simulink model "s_c107m32k_vlbi"  (R2018a)
settings: Solver=VariableStepDiscrete  StartTime=0.0  StopTime=(2^15)*10  RelTol=1e-3
undefined symbols (not defined in the file): fft_stages, n_bits_xengs
libraries: xbsIndex_r4 x23049, casper_library_misc x45, xps_library x4, casper_library_scopes x3, simulink x2
(part 151 of 201)

== system s_c107m32k_vlbi/cd_hmc/hmc_delay/ctrl_pol0/add_parity ==
  din : Inport
  Concat : xbsIndex_r4/Concat  num_inputs=2  dbl_ovrd=off  block_type=concat
  Delay1 : xbsIndex_r4/Delay  rst=off  infoeditControl=Selection of Reset will increase slice count due to use of real FFs and instead of SRLs  en=off  latency=3  reg_retiming=on  dbl_ovrd=off  block_type=delay
  Delay2 : xbsIndex_r4/Delay  rst=off  infoeditControl=Selection of Reset will increase slice count due to use of real FFs and instead of SRLs  en=off  latency=1  reg_retiming=on  dbl_ovrd=off  block_type=delay
  bus_expand : Subsystem  AncestorBlock=casper_library_flow_control/bus_expand  mask(bus_expand){mode=divisions of equal size, outputNum=80, outputWidth=1, outputBinaryPt=0, outputArithmeticType=0, show_format=off, outputToWorkspace=off, variablePrefix=out, outputToModelAsWell=on}
      mask prompts: outputNum "Number of outputs:"; outputWidth "Output width:"; outputBinaryPt "Output binary point position:"; outputArithmeticType "Output arithmetic type (ufix=0, fix=1, bool=2):"; show_format "Print format string?"; outputToWorkspace "Output to workspace?"; variablePrefix "Variable name prefix:"; outputToModelAsWell "Output to model as well?"
      mask help:
      | Expands a 'bus' made using a bus_create or Xilinx
      | concat block.
      | The input will be divided into the specified number
      | of outputs with the specified arithmetic types.
      | Divisions are made from most significant bit.
      mask init: same as s_c107m32k_vlbi/bus_expand1
      settings: AttributesFormatString=80 outputs
      mask TypeOptions mode: divisions of equal size | divisions of arbitrary size
      mask Callback mode: bus_expand_callback();
      mask Callback outputWidth: bus_expand_callback();
      mask Callback outputToWorkspace: bus_expand_callback();
  parity : xbsIndex_r4/Logical  logical_function=XOR  inputs=80  en=off  latency=3  precision=Full  arith_type=Unsigned  n_bits=16  bin_pt=0  align_bp=on  dbl_ovrd=off  block_type=logical
  dout : Outport
  wires:
  Concat/1 -> dout/1
  parity/1 -> Concat/1
  Delay1/1 -> Concat/2
  din/1 -> Delay2/1
  bus_expand/70(out11) -> parity/70
  bus_expand/8(out73) -> parity/8
  bus_expand/31(out50) -> parity/31
  bus_expand/24(out57) -> parity/24
  bus_expand/30(out51) -> parity/30
  bus_expand/38(out43) -> parity/38
  bus_expand/61(out20) -> parity/61
  bus_expand/50(out31) -> parity/50
  bus_expand/77(out4) -> parity/77
  bus_expand/4(out77) -> parity/4
  bus_expand/68(out13) -> parity/68
  bus_expand/59(out22) -> parity/59
  bus_expand/65(out16) -> parity/65
  bus_expand/14(out67) -> parity/14
  bus_expand/7(out74) -> parity/7
  bus_expand/44(out37) -> parity/44
  bus_expand/43(out38) -> parity/43
  bus_expand/23(out58) -> parity/23
  bus_expand/22(out59) -> parity/22
  bus_expand/67(out14) -> parity/67
  bus_expand/2(out79) -> parity/2
  bus_expand/48(out33) -> parity/48
  bus_expand/42(out39) -> parity/42
  bus_expand/78(out3) -> parity/78
  bus_expand/58(out23) -> parity/58
  bus_expand/80(lsb_out1) -> parity/80
  bus_expand/72(out9) -> parity/72
  bus_expand/18(out63) -> parity/18
  bus_expand/15(out66) -> parity/15
  bus_expand/17(out64) -> parity/17
  bus_expand/1(msb_out80) -> parity/1
  bus_expand/6(out75) -> parity/6
  bus_expand/47(out34) -> parity/47
  bus_expand/37(out44) -> parity/37
  bus_expand/71(out10) -> parity/71
  bus_expand/73(out8) -> parity/73
  bus_expand/51(out30) -> parity/51
  bus_expand/21(out60) -> parity/21
  bus_expand/13(out68) -> parity/13
  bus_expand/20(out61) -> parity/20
  bus_expand/76(out5) -> parity/76
  bus_expand/57(out24) -> parity/57
  bus_expand/63(out18) -> parity/63
  bus_expand/33(out48) -> parity/33
  bus_expand/75(out6) -> parity/75
  bus_expand/60(out21) -> parity/60
  bus_expand/54(out27) -> parity/54
  bus_expand/28(out53) -> parity/28
  bus_expand/69(out12) -> parity/69
  bus_expand/10(out71) -> parity/10
  bus_expand/32(out49) -> parity/32
  bus_expand/62(out19) -> parity/62
  bus_expand/36(out45) -> parity/36
  bus_expand/64(out17) -> parity/64
  bus_expand/46(out35) -> parity/46
  bus_expand/3(out78) -> parity/3
  bus_expand/56(out25) -> parity/56
  bus_expand/5(out76) -> parity/5
  bus_expand/19(out62) -> parity/19
  bus_expand/74(out7) -> parity/74
  bus_expand/25(out56) -> parity/25
  bus_expand/49(out32) -> parity/49
  bus_expand/11(out70) -> parity/11
  bus_expand/52(out29) -> parity/52
  bus_expand/41(out40) -> parity/41
  bus_expand/79(out2) -> parity/79
  bus_expand/27(out54) -> parity/27
  bus_expand/29(out52) -> parity/29
  bus_expand/26(out55) -> parity/26
  bus_expand/45(out36) -> parity/45
  bus_expand/34(out47) -> parity/34
  bus_expand/12(out69) -> parity/12
  bus_expand/16(out65) -> parity/16
  bus_expand/9(out72) -> parity/9
  bus_expand/55(out26) -> parity/55
  bus_expand/40(out41) -> parity/40
  bus_expand/35(out46) -> parity/35
  bus_expand/39(out42) -> parity/39
  bus_expand/66(out15) -> parity/66
  bus_expand/53(out28) -> parity/53
  Delay2/1 -> Delay1/1, bus_expand/1(bus_in)

== system s_c107m32k_vlbi/cd_hmc/hmc_delay/ctrl_pol1/add_parity ==
  din : Inport
  Concat : xbsIndex_r4/Concat  num_inputs=2  dbl_ovrd=off  block_type=concat
  Delay1 : xbsIndex_r4/Delay  rst=off  infoeditControl=Selection of Reset will increase slice count due to use of real FFs and instead of SRLs  en=off  latency=3  reg_retiming=on  dbl_ovrd=off  block_type=delay
  Delay2 : xbsIndex_r4/Delay  rst=off  infoeditControl=Selection of Reset will increase slice count due to use of real FFs and instead of SRLs  en=off  latency=1  reg_retiming=on  dbl_ovrd=off  block_type=delay
  bus_expand : Subsystem  AncestorBlock=casper_library_flow_control/bus_expand  mask(bus_expand){mode=divisions of equal size, outputNum=80, outputWidth=1, outputBinaryPt=0, outputArithmeticType=0, show_format=off, outputToWorkspace=off, variablePrefix=out, outputToModelAsWell=on}
      mask prompts: outputNum "Number of outputs:"; outputWidth "Output width:"; outputBinaryPt "Output binary point position:"; outputArithmeticType "Output arithmetic type (ufix=0, fix=1, bool=2):"; show_format "Print format string?"; outputToWorkspace "Output to workspace?"; variablePrefix "Variable name prefix:"; outputToModelAsWell "Output to model as well?"
      mask help:
      | Expands a 'bus' made using a bus_create or Xilinx
      | concat block.
      | The input will be divided into the specified number
      | of outputs with the specified arithmetic types.
      | Divisions are made from most significant bit.
      mask init: same as s_c107m32k_vlbi/bus_expand1
      settings: AttributesFormatString=80 outputs
      mask TypeOptions mode: divisions of equal size | divisions of arbitrary size
      mask Callback mode: bus_expand_callback();
      mask Callback outputWidth: bus_expand_callback();
      mask Callback outputToWorkspace: bus_expand_callback();
  parity : xbsIndex_r4/Logical  logical_function=XOR  inputs=80  en=off  latency=3  precision=Full  arith_type=Unsigned  n_bits=16  bin_pt=0  align_bp=on  dbl_ovrd=off  block_type=logical
  dout : Outport
  wires:
  Concat/1 -> dout/1
  parity/1 -> Concat/1
  Delay1/1 -> Concat/2
  din/1 -> Delay2/1
  bus_expand/70(out11) -> parity/70
  bus_expand/8(out73) -> parity/8
  bus_expand/31(out50) -> parity/31
  bus_expand/24(out57) -> parity/24
  bus_expand/30(out51) -> parity/30
  bus_expand/38(out43) -> parity/38
  bus_expand/61(out20) -> parity/61
  bus_expand/50(out31) -> parity/50
  bus_expand/77(out4) -> parity/77
  bus_expand/4(out77) -> parity/4
  bus_expand/68(out13) -> parity/68
  bus_expand/59(out22) -> parity/59
  bus_expand/65(out16) -> parity/65
  bus_expand/14(out67) -> parity/14
  bus_expand/7(out74) -> parity/7
  bus_expand/44(out37) -> parity/44
  bus_expand/43(out38) -> parity/43
  bus_expand/23(out58) -> parity/23
  bus_expand/22(out59) -> parity/22
  bus_expand/67(out14) -> parity/67
  bus_expand/2(out79) -> parity/2
  bus_expand/48(out33) -> parity/48
  bus_expand/42(out39) -> parity/42
  bus_expand/78(out3) -> parity/78
  bus_expand/58(out23) -> parity/58
  bus_expand/80(lsb_out1) -> parity/80
  bus_expand/72(out9) -> parity/72
  bus_expand/18(out63) -> parity/18
  bus_expand/15(out66) -> parity/15
  bus_expand/17(out64) -> parity/17
  bus_expand/1(msb_out80) -> parity/1
  bus_expand/6(out75) -> parity/6
  bus_expand/47(out34) -> parity/47
  bus_expand/37(out44) -> parity/37
  bus_expand/71(out10) -> parity/71
  bus_expand/73(out8) -> parity/73
  bus_expand/51(out30) -> parity/51
  bus_expand/21(out60) -> parity/21
  bus_expand/13(out68) -> parity/13
  bus_expand/20(out61) -> parity/20
  bus_expand/76(out5) -> parity/76
  bus_expand/57(out24) -> parity/57
  bus_expand/63(out18) -> parity/63
  bus_expand/33(out48) -> parity/33
  bus_expand/75(out6) -> parity/75
  bus_expand/60(out21) -> parity/60
  bus_expand/54(out27) -> parity/54
  bus_expand/28(out53) -> parity/28
  bus_expand/69(out12) -> parity/69
  bus_expand/10(out71) -> parity/10
  bus_expand/32(out49) -> parity/32
  bus_expand/62(out19) -> parity/62
  bus_expand/36(out45) -> parity/36
  bus_expand/64(out17) -> parity/64
  bus_expand/46(out35) -> parity/46
  bus_expand/3(out78) -> parity/3
  bus_expand/56(out25) -> parity/56
  bus_expand/5(out76) -> parity/5
  bus_expand/19(out62) -> parity/19
  bus_expand/74(out7) -> parity/74
  bus_expand/25(out56) -> parity/25
  bus_expand/49(out32) -> parity/49
  bus_expand/11(out70) -> parity/11
  bus_expand/52(out29) -> parity/52
  bus_expand/41(out40) -> parity/41
  bus_expand/79(out2) -> parity/79
  bus_expand/27(out54) -> parity/27
  bus_expand/29(out52) -> parity/29
  bus_expand/26(out55) -> parity/26
  bus_expand/45(out36) -> parity/45
  bus_expand/34(out47) -> parity/34
  bus_expand/12(out69) -> parity/12
  bus_expand/16(out65) -> parity/16
  bus_expand/9(out72) -> parity/9
  bus_expand/55(out26) -> parity/55
  bus_expand/40(out41) -> parity/40
  bus_expand/35(out46) -> parity/35
  bus_expand/39(out42) -> parity/39
  bus_expand/66(out15) -> parity/66
  bus_expand/53(out28) -> parity/53
  Delay2/1 -> Delay1/1, bus_expand/1(bus_in)

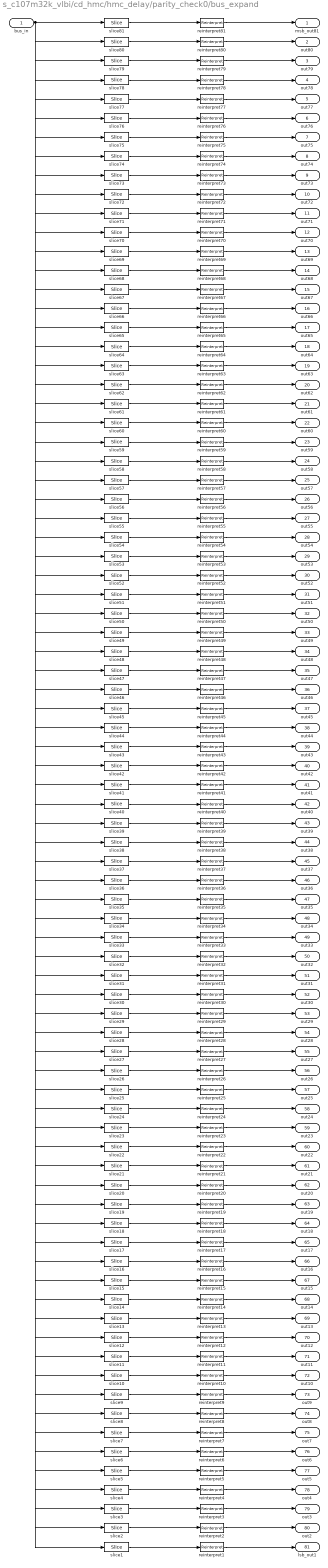
== system s_c107m32k_vlbi/cd_hmc/hmc_delay/parity_check0/bus_expand ==
  bus_in : Inport
  reinterpret{1..81} (81 alike) : xbsIndex_r4/Reinterpret  force_arith_type=on  arith_type=Unsigned  force_bin_pt=on  bin_pt=0  block_type=reinterpret
  slice1 : xbsIndex_r4/Slice  nbits=1  boolean_output=off  mode=Upper Bit Location + Width  bit1=-80  base1=MSB of Input  bit0=0  base0=LSB of Input  dbl_ovrd=off  block_type=slice
  slice10 : xbsIndex_r4/Slice  nbits=1  boolean_output=off  mode=Upper Bit Location + Width  bit1=-71  base1=MSB of Input  bit0=0  base0=LSB of Input  dbl_ovrd=off  block_type=slice
  slice11 : xbsIndex_r4/Slice  nbits=1  boolean_output=off  mode=Upper Bit Location + Width  bit1=-70  base1=MSB of Input  bit0=0  base0=LSB of Input  dbl_ovrd=off  block_type=slice
  slice12 : xbsIndex_r4/Slice  nbits=1  boolean_output=off  mode=Upper Bit Location + Width  bit1=-69  base1=MSB of Input  bit0=0  base0=LSB of Input  dbl_ovrd=off  block_type=slice
  slice13 : xbsIndex_r4/Slice  nbits=1  boolean_output=off  mode=Upper Bit Location + Width  bit1=-68  base1=MSB of Input  bit0=0  base0=LSB of Input  dbl_ovrd=off  block_type=slice
  slice14 : xbsIndex_r4/Slice  nbits=1  boolean_output=off  mode=Upper Bit Location + Width  bit1=-67  base1=MSB of Input  bit0=0  base0=LSB of Input  dbl_ovrd=off  block_type=slice
  slice15 : xbsIndex_r4/Slice  nbits=1  boolean_output=off  mode=Upper Bit Location + Width  bit1=-66  base1=MSB of Input  bit0=0  base0=LSB of Input  dbl_ovrd=off  block_type=slice
  slice16 : xbsIndex_r4/Slice  nbits=1  boolean_output=off  mode=Upper Bit Location + Width  bit1=-65  base1=MSB of Input  bit0=0  base0=LSB of Input  dbl_ovrd=off  block_type=slice
  slice17 : xbsIndex_r4/Slice  nbits=1  boolean_output=off  mode=Upper Bit Location + Width  bit1=-64  base1=MSB of Input  bit0=0  base0=LSB of Input  dbl_ovrd=off  block_type=slice
  slice18 : xbsIndex_r4/Slice  nbits=1  boolean_output=off  mode=Upper Bit Location + Width  bit1=-63  base1=MSB of Input  bit0=0  base0=LSB of Input  dbl_ovrd=off  block_type=slice
  slice19 : xbsIndex_r4/Slice  nbits=1  boolean_output=off  mode=Upper Bit Location + Width  bit1=-62  base1=MSB of Input  bit0=0  base0=LSB of Input  dbl_ovrd=off  block_type=slice
  slice2 : xbsIndex_r4/Slice  nbits=1  boolean_output=off  mode=Upper Bit Location + Width  bit1=-79  base1=MSB of Input  bit0=0  base0=LSB of Input  dbl_ovrd=off  block_type=slice
  slice20 : xbsIndex_r4/Slice  nbits=1  boolean_output=off  mode=Upper Bit Location + Width  bit1=-61  base1=MSB of Input  bit0=0  base0=LSB of Input  dbl_ovrd=off  block_type=slice
  slice21 : xbsIndex_r4/Slice  nbits=1  boolean_output=off  mode=Upper Bit Location + Width  bit1=-60  base1=MSB of Input  bit0=0  base0=LSB of Input  dbl_ovrd=off  block_type=slice
  slice22 : xbsIndex_r4/Slice  nbits=1  boolean_output=off  mode=Upper Bit Location + Width  bit1=-59  base1=MSB of Input  bit0=0  base0=LSB of Input  dbl_ovrd=off  block_type=slice
  slice23 : xbsIndex_r4/Slice  nbits=1  boolean_output=off  mode=Upper Bit Location + Width  bit1=-58  base1=MSB of Input  bit0=0  base0=LSB of Input  dbl_ovrd=off  block_type=slice
  slice24 : xbsIndex_r4/Slice  nbits=1  boolean_output=off  mode=Upper Bit Location + Width  bit1=-57  base1=MSB of Input  bit0=0  base0=LSB of Input  dbl_ovrd=off  block_type=slice
  slice25 : xbsIndex_r4/Slice  nbits=1  boolean_output=off  mode=Upper Bit Location + Width  bit1=-56  base1=MSB of Input  bit0=0  base0=LSB of Input  dbl_ovrd=off  block_type=slice
  slice26 : xbsIndex_r4/Slice  nbits=1  boolean_output=off  mode=Upper Bit Location + Width  bit1=-55  base1=MSB of Input  bit0=0  base0=LSB of Input  dbl_ovrd=off  block_type=slice
  slice27 : xbsIndex_r4/Slice  nbits=1  boolean_output=off  mode=Upper Bit Location + Width  bit1=-54  base1=MSB of Input  bit0=0  base0=LSB of Input  dbl_ovrd=off  block_type=slice
  slice28 : xbsIndex_r4/Slice  nbits=1  boolean_output=off  mode=Upper Bit Location + Width  bit1=-53  base1=MSB of Input  bit0=0  base0=LSB of Input  dbl_ovrd=off  block_type=slice
  slice29 : xbsIndex_r4/Slice  nbits=1  boolean_output=off  mode=Upper Bit Location + Width  bit1=-52  base1=MSB of Input  bit0=0  base0=LSB of Input  dbl_ovrd=off  block_type=slice
  slice3 : xbsIndex_r4/Slice  nbits=1  boolean_output=off  mode=Upper Bit Location + Width  bit1=-78  base1=MSB of Input  bit0=0  base0=LSB of Input  dbl_ovrd=off  block_type=slice
  slice30 : xbsIndex_r4/Slice  nbits=1  boolean_output=off  mode=Upper Bit Location + Width  bit1=-51  base1=MSB of Input  bit0=0  base0=LSB of Input  dbl_ovrd=off  block_type=slice
  slice31 : xbsIndex_r4/Slice  nbits=1  boolean_output=off  mode=Upper Bit Location + Width  bit1=-50  base1=MSB of Input  bit0=0  base0=LSB of Input  dbl_ovrd=off  block_type=slice
  slice32 : xbsIndex_r4/Slice  nbits=1  boolean_output=off  mode=Upper Bit Location + Width  bit1=-49  base1=MSB of Input  bit0=0  base0=LSB of Input  dbl_ovrd=off  block_type=slice
  slice33 : xbsIndex_r4/Slice  nbits=1  boolean_output=off  mode=Upper Bit Location + Width  bit1=-48  base1=MSB of Input  bit0=0  base0=LSB of Input  dbl_ovrd=off  block_type=slice
  slice34 : xbsIndex_r4/Slice  nbits=1  boolean_output=off  mode=Upper Bit Location + Width  bit1=-47  base1=MSB of Input  bit0=0  base0=LSB of Input  dbl_ovrd=off  block_type=slice
  slice35 : xbsIndex_r4/Slice  nbits=1  boolean_output=off  mode=Upper Bit Location + Width  bit1=-46  base1=MSB of Input  bit0=0  base0=LSB of Input  dbl_ovrd=off  block_type=slice
  slice36 : xbsIndex_r4/Slice  nbits=1  boolean_output=off  mode=Upper Bit Location + Width  bit1=-45  base1=MSB of Input  bit0=0  base0=LSB of Input  dbl_ovrd=off  block_type=slice
  slice37 : xbsIndex_r4/Slice  nbits=1  boolean_output=off  mode=Upper Bit Location + Width  bit1=-44  base1=MSB of Input  bit0=0  base0=LSB of Input  dbl_ovrd=off  block_type=slice
  slice38 : xbsIndex_r4/Slice  nbits=1  boolean_output=off  mode=Upper Bit Location + Width  bit1=-43  base1=MSB of Input  bit0=0  base0=LSB of Input  dbl_ovrd=off  block_type=slice
  slice39 : xbsIndex_r4/Slice  nbits=1  boolean_output=off  mode=Upper Bit Location + Width  bit1=-42  base1=MSB of Input  bit0=0  base0=LSB of Input  dbl_ovrd=off  block_type=slice
  slice4 : xbsIndex_r4/Slice  nbits=1  boolean_output=off  mode=Upper Bit Location + Width  bit1=-77  base1=MSB of Input  bit0=0  base0=LSB of Input  dbl_ovrd=off  block_type=slice
  slice40 : xbsIndex_r4/Slice  nbits=1  boolean_output=off  mode=Upper Bit Location + Width  bit1=-41  base1=MSB of Input  bit0=0  base0=LSB of Input  dbl_ovrd=off  block_type=slice
  slice41 : xbsIndex_r4/Slice  nbits=1  boolean_output=off  mode=Upper Bit Location + Width  bit1=-40  base1=MSB of Input  bit0=0  base0=LSB of Input  dbl_ovrd=off  block_type=slice
  slice42 : xbsIndex_r4/Slice  nbits=1  boolean_output=off  mode=Upper Bit Location + Width  bit1=-39  base1=MSB of Input  bit0=0  base0=LSB of Input  dbl_ovrd=off  block_type=slice
  slice43 : xbsIndex_r4/Slice  nbits=1  boolean_output=off  mode=Upper Bit Location + Width  bit1=-38  base1=MSB of Input  bit0=0  base0=LSB of Input  dbl_ovrd=off  block_type=slice
  slice44 : xbsIndex_r4/Slice  nbits=1  boolean_output=off  mode=Upper Bit Location + Width  bit1=-37  base1=MSB of Input  bit0=0  base0=LSB of Input  dbl_ovrd=off  block_type=slice
  slice45 : xbsIndex_r4/Slice  nbits=1  boolean_output=off  mode=Upper Bit Location + Width  bit1=-36  base1=MSB of Input  bit0=0  base0=LSB of Input  dbl_ovrd=off  block_type=slice
  slice46 : xbsIndex_r4/Slice  nbits=1  boolean_output=off  mode=Upper Bit Location + Width  bit1=-35  base1=MSB of Input  bit0=0  base0=LSB of Input  dbl_ovrd=off  block_type=slice
  slice47 : xbsIndex_r4/Slice  nbits=1  boolean_output=off  mode=Upper Bit Location + Width  bit1=-34  base1=MSB of Input  bit0=0  base0=LSB of Input  dbl_ovrd=off  block_type=slice
  slice48 : xbsIndex_r4/Slice  nbits=1  boolean_output=off  mode=Upper Bit Location + Width  bit1=-33  base1=MSB of Input  bit0=0  base0=LSB of Input  dbl_ovrd=off  block_type=slice
  slice49 : xbsIndex_r4/Slice  nbits=1  boolean_output=off  mode=Upper Bit Location + Width  bit1=-32  base1=MSB of Input  bit0=0  base0=LSB of Input  dbl_ovrd=off  block_type=slice
  slice5 : xbsIndex_r4/Slice  nbits=1  boolean_output=off  mode=Upper Bit Location + Width  bit1=-76  base1=MSB of Input  bit0=0  base0=LSB of Input  dbl_ovrd=off  block_type=slice
  slice50 : xbsIndex_r4/Slice  nbits=1  boolean_output=off  mode=Upper Bit Location + Width  bit1=-31  base1=MSB of Input  bit0=0  base0=LSB of Input  dbl_ovrd=off  block_type=slice
  slice51 : xbsIndex_r4/Slice  nbits=1  boolean_output=off  mode=Upper Bit Location + Width  bit1=-30  base1=MSB of Input  bit0=0  base0=LSB of Input  dbl_ovrd=off  block_type=slice
  slice52 : xbsIndex_r4/Slice  nbits=1  boolean_output=off  mode=Upper Bit Location + Width  bit1=-29  base1=MSB of Input  bit0=0  base0=LSB of Input  dbl_ovrd=off  block_type=slice
  slice53 : xbsIndex_r4/Slice  nbits=1  boolean_output=off  mode=Upper Bit Location + Width  bit1=-28  base1=MSB of Input  bit0=0  base0=LSB of Input  dbl_ovrd=off  block_type=slice
  slice54 : xbsIndex_r4/Slice  nbits=1  boolean_output=off  mode=Upper Bit Location + Width  bit1=-27  base1=MSB of Input  bit0=0  base0=LSB of Input  dbl_ovrd=off  block_type=slice
  slice55 : xbsIndex_r4/Slice  nbits=1  boolean_output=off  mode=Upper Bit Location + Width  bit1=-26  base1=MSB of Input  bit0=0  base0=LSB of Input  dbl_ovrd=off  block_type=slice
  slice56 : xbsIndex_r4/Slice  nbits=1  boolean_output=off  mode=Upper Bit Location + Width  bit1=-25  base1=MSB of Input  bit0=0  base0=LSB of Input  dbl_ovrd=off  block_type=slice
  slice57 : xbsIndex_r4/Slice  nbits=1  boolean_output=off  mode=Upper Bit Location + Width  bit1=-24  base1=MSB of Input  bit0=0  base0=LSB of Input  dbl_ovrd=off  block_type=slice
  slice58 : xbsIndex_r4/Slice  nbits=1  boolean_output=off  mode=Upper Bit Location + Width  bit1=-23  base1=MSB of Input  bit0=0  base0=LSB of Input  dbl_ovrd=off  block_type=slice
  slice59 : xbsIndex_r4/Slice  nbits=1  boolean_output=off  mode=Upper Bit Location + Width  bit1=-22  base1=MSB of Input  bit0=0  base0=LSB of Input  dbl_ovrd=off  block_type=slice
  slice6 : xbsIndex_r4/Slice  nbits=1  boolean_output=off  mode=Upper Bit Location + Width  bit1=-75  base1=MSB of Input  bit0=0  base0=LSB of Input  dbl_ovrd=off  block_type=slice
  slice60 : xbsIndex_r4/Slice  nbits=1  boolean_output=off  mode=Upper Bit Location + Width  bit1=-21  base1=MSB of Input  bit0=0  base0=LSB of Input  dbl_ovrd=off  block_type=slice
  slice61 : xbsIndex_r4/Slice  nbits=1  boolean_output=off  mode=Upper Bit Location + Width  bit1=-20  base1=MSB of Input  bit0=0  base0=LSB of Input  dbl_ovrd=off  block_type=slice
  slice62 : xbsIndex_r4/Slice  nbits=1  boolean_output=off  mode=Upper Bit Location + Width  bit1=-19  base1=MSB of Input  bit0=0  base0=LSB of Input  dbl_ovrd=off  block_type=slice
  slice63 : xbsIndex_r4/Slice  nbits=1  boolean_output=off  mode=Upper Bit Location + Width  bit1=-18  base1=MSB of Input  bit0=0  base0=LSB of Input  dbl_ovrd=off  block_type=slice
  slice64 : xbsIndex_r4/Slice  nbits=1  boolean_output=off  mode=Upper Bit Location + Width  bit1=-17  base1=MSB of Input  bit0=0  base0=LSB of Input  dbl_ovrd=off  block_type=slice
  slice65 : xbsIndex_r4/Slice  nbits=1  boolean_output=off  mode=Upper Bit Location + Width  bit1=-16  base1=MSB of Input  bit0=0  base0=LSB of Input  dbl_ovrd=off  block_type=slice
  slice66 : xbsIndex_r4/Slice  nbits=1  boolean_output=off  mode=Upper Bit Location + Width  bit1=-15  base1=MSB of Input  bit0=0  base0=LSB of Input  dbl_ovrd=off  block_type=slice
  slice67 : xbsIndex_r4/Slice  nbits=1  boolean_output=off  mode=Upper Bit Location + Width  bit1=-14  base1=MSB of Input  bit0=0  base0=LSB of Input  dbl_ovrd=off  block_type=slice
  slice68 : xbsIndex_r4/Slice  nbits=1  boolean_output=off  mode=Upper Bit Location + Width  bit1=-13  base1=MSB of Input  bit0=0  base0=LSB of Input  dbl_ovrd=off  block_type=slice
  slice69 : xbsIndex_r4/Slice  nbits=1  boolean_output=off  mode=Upper Bit Location + Width  bit1=-12  base1=MSB of Input  bit0=0  base0=LSB of Input  dbl_ovrd=off  block_type=slice
  slice7 : xbsIndex_r4/Slice  nbits=1  boolean_output=off  mode=Upper Bit Location + Width  bit1=-74  base1=MSB of Input  bit0=0  base0=LSB of Input  dbl_ovrd=off  block_type=slice
  slice70 : xbsIndex_r4/Slice  nbits=1  boolean_output=off  mode=Upper Bit Location + Width  bit1=-11  base1=MSB of Input  bit0=0  base0=LSB of Input  dbl_ovrd=off  block_type=slice
  slice71 : xbsIndex_r4/Slice  nbits=1  boolean_output=off  mode=Upper Bit Location + Width  bit1=-10  base1=MSB of Input  bit0=0  base0=LSB of Input  dbl_ovrd=off  block_type=slice
  slice72 : xbsIndex_r4/Slice  nbits=1  boolean_output=off  mode=Upper Bit Location + Width  bit1=-9  base1=MSB of Input  bit0=0  base0=LSB of Input  dbl_ovrd=off  block_type=slice
  slice73 : xbsIndex_r4/Slice  nbits=1  boolean_output=off  mode=Upper Bit Location + Width  bit1=-8  base1=MSB of Input  bit0=0  base0=LSB of Input  dbl_ovrd=off  block_type=slice
  slice74 : xbsIndex_r4/Slice  nbits=1  boolean_output=off  mode=Upper Bit Location + Width  bit1=-7  base1=MSB of Input  bit0=0  base0=LSB of Input  dbl_ovrd=off  block_type=slice
  slice75 : xbsIndex_r4/Slice  nbits=1  boolean_output=off  mode=Upper Bit Location + Width  bit1=-6  base1=MSB of Input  bit0=0  base0=LSB of Input  dbl_ovrd=off  block_type=slice
  slice76 : xbsIndex_r4/Slice  nbits=1  boolean_output=off  mode=Upper Bit Location + Width  bit1=-5  base1=MSB of Input  bit0=0  base0=LSB of Input  dbl_ovrd=off  block_type=slice
  slice77 : xbsIndex_r4/Slice  nbits=1  boolean_output=off  mode=Upper Bit Location + Width  bit1=-4  base1=MSB of Input  bit0=0  base0=LSB of Input  dbl_ovrd=off  block_type=slice
  slice78 : xbsIndex_r4/Slice  nbits=1  boolean_output=off  mode=Upper Bit Location + Width  bit1=-3  base1=MSB of Input  bit0=0  base0=LSB of Input  dbl_ovrd=off  block_type=slice
  slice79 : xbsIndex_r4/Slice  nbits=1  boolean_output=off  mode=Upper Bit Location + Width  bit1=-2  base1=MSB of Input  bit0=0  base0=LSB of Input  dbl_ovrd=off  block_type=slice
  slice8 : xbsIndex_r4/Slice  nbits=1  boolean_output=off  mode=Upper Bit Location + Width  bit1=-73  base1=MSB of Input  bit0=0  base0=LSB of Input  dbl_ovrd=off  block_type=slice
  slice80 : xbsIndex_r4/Slice  nbits=1  boolean_output=off  mode=Upper Bit Location + Width  bit1=-1  base1=MSB of Input  bit0=0  base0=LSB of Input  dbl_ovrd=off  block_type=slice
  slice81 : xbsIndex_r4/Slice  nbits=1  boolean_output=off  mode=Upper Bit Location + Width  bit1=0  base1=MSB of Input  bit0=0  base0=LSB of Input  dbl_ovrd=off  block_type=slice
  slice9 : xbsIndex_r4/Slice  nbits=1  boolean_output=off  mode=Upper Bit Location + Width  bit1=-72  base1=MSB of Input  bit0=0  base0=LSB of Input  dbl_ovrd=off  block_type=slice
  msb_out81 : Outport
  out80 : Outport  Port=2
  out79 : Outport  Port=3
  out78 : Outport  Port=4
  out77 : Outport  Port=5
  out76 : Outport  Port=6
  out75 : Outport  Port=7
  out74 : Outport  Port=8
  out73 : Outport  Port=9
  out72 : Outport  Port=10
  out71 : Outport  Port=11
  out70 : Outport  Port=12
  out69 : Outport  Port=13
  out68 : Outport  Port=14
  out67 : Outport  Port=15
  out66 : Outport  Port=16
  out65 : Outport  Port=17
  out64 : Outport  Port=18
  out63 : Outport  Port=19
  out62 : Outport  Port=20
  out61 : Outport  Port=21
  out60 : Outport  Port=22
  out59 : Outport  Port=23
  out58 : Outport  Port=24
  out57 : Outport  Port=25
  out56 : Outport  Port=26
  out55 : Outport  Port=27
  out54 : Outport  Port=28
  out53 : Outport  Port=29
  out52 : Outport  Port=30
  out51 : Outport  Port=31
  out50 : Outport  Port=32
  out49 : Outport  Port=33
  out48 : Outport  Port=34
  out47 : Outport  Port=35
  out46 : Outport  Port=36
  out45 : Outport  Port=37
  out44 : Outport  Port=38
  out43 : Outport  Port=39
  out42 : Outport  Port=40
  out41 : Outport  Port=41
  out40 : Outport  Port=42
  out39 : Outport  Port=43
  out38 : Outport  Port=44
  out37 : Outport  Port=45
  out36 : Outport  Port=46
  out35 : Outport  Port=47
  out34 : Outport  Port=48
  out33 : Outport  Port=49
  out32 : Outport  Port=50
  out31 : Outport  Port=51
  out30 : Outport  Port=52
  out29 : Outport  Port=53
  out28 : Outport  Port=54
  out27 : Outport  Port=55
  out26 : Outport  Port=56
  out25 : Outport  Port=57
  out24 : Outport  Port=58
  out23 : Outport  Port=59
  out22 : Outport  Port=60
  out21 : Outport  Port=61
  out20 : Outport  Port=62
  out19 : Outport  Port=63
  out18 : Outport  Port=64
  out17 : Outport  Port=65
  out16 : Outport  Port=66
  out15 : Outport  Port=67
  out14 : Outport  Port=68
  out13 : Outport  Port=69
  out12 : Outport  Port=70
  out11 : Outport  Port=71
  out10 : Outport  Port=72
  out9 : Outport  Port=73
  out8 : Outport  Port=74
  out7 : Outport  Port=75
  out6 : Outport  Port=76
  out5 : Outport  Port=77
  out4 : Outport  Port=78
  out3 : Outport  Port=79
  out2 : Outport  Port=80
  lsb_out1 : Outport  Port=81
  wires:
  reinterpret1/1 -> lsb_out1/1
  slice1/1 -> reinterpret1/1
  reinterpret2/1 -> out2/1
  slice2/1 -> reinterpret2/1
  reinterpret3/1 -> out3/1
  slice3/1 -> reinterpret3/1
  reinterpret4/1 -> out4/1
  slice4/1 -> reinterpret4/1
  reinterpret5/1 -> out5/1
  slice5/1 -> reinterpret5/1
  reinterpret6/1 -> out6/1
  slice6/1 -> reinterpret6/1
  reinterpret7/1 -> out7/1
  slice7/1 -> reinterpret7/1
  reinterpret8/1 -> out8/1
  slice8/1 -> reinterpret8/1
  reinterpret9/1 -> out9/1
  slice9/1 -> reinterpret9/1
  reinterpret10/1 -> out10/1
  slice10/1 -> reinterpret10/1
  reinterpret11/1 -> out11/1
  slice11/1 -> reinterpret11/1
  reinterpret12/1 -> out12/1
  slice12/1 -> reinterpret12/1
  reinterpret13/1 -> out13/1
  slice13/1 -> reinterpret13/1
  reinterpret14/1 -> out14/1
  slice14/1 -> reinterpret14/1
  reinterpret15/1 -> out15/1
  slice15/1 -> reinterpret15/1
  reinterpret16/1 -> out16/1
  slice16/1 -> reinterpret16/1
  reinterpret17/1 -> out17/1
  slice17/1 -> reinterpret17/1
  reinterpret18/1 -> out18/1
  slice18/1 -> reinterpret18/1
  reinterpret19/1 -> out19/1
  slice19/1 -> reinterpret19/1
  reinterpret20/1 -> out20/1
  slice20/1 -> reinterpret20/1
  reinterpret21/1 -> out21/1
  slice21/1 -> reinterpret21/1
  reinterpret22/1 -> out22/1
  slice22/1 -> reinterpret22/1
  reinterpret23/1 -> out23/1
  slice23/1 -> reinterpret23/1
  reinterpret24/1 -> out24/1
  slice24/1 -> reinterpret24/1
  reinterpret25/1 -> out25/1
  slice25/1 -> reinterpret25/1
  reinterpret26/1 -> out26/1
  slice26/1 -> reinterpret26/1
  reinterpret27/1 -> out27/1
  slice27/1 -> reinterpret27/1
  reinterpret28/1 -> out28/1
  slice28/1 -> reinterpret28/1
  reinterpret29/1 -> out29/1
  slice29/1 -> reinterpret29/1
  reinterpret30/1 -> out30/1
  slice30/1 -> reinterpret30/1
  reinterpret31/1 -> out31/1
  slice31/1 -> reinterpret31/1
  reinterpret32/1 -> out32/1
  slice32/1 -> reinterpret32/1
  reinterpret33/1 -> out33/1
  slice33/1 -> reinterpret33/1
  reinterpret34/1 -> out34/1
  slice34/1 -> reinterpret34/1
  reinterpret35/1 -> out35/1
  slice35/1 -> reinterpret35/1
  reinterpret36/1 -> out36/1
  slice36/1 -> reinterpret36/1
  reinterpret37/1 -> out37/1
  slice37/1 -> reinterpret37/1
  reinterpret38/1 -> out38/1
  slice38/1 -> reinterpret38/1
  reinterpret39/1 -> out39/1
  slice39/1 -> reinterpret39/1
  reinterpret40/1 -> out40/1
  slice40/1 -> reinterpret40/1
  reinterpret41/1 -> out41/1
  slice41/1 -> reinterpret41/1
  reinterpret42/1 -> out42/1
  slice42/1 -> reinterpret42/1
  reinterpret43/1 -> out43/1
  slice43/1 -> reinterpret43/1
  reinterpret44/1 -> out44/1
  slice44/1 -> reinterpret44/1
  reinterpret45/1 -> out45/1
  slice45/1 -> reinterpret45/1
  reinterpret46/1 -> out46/1
  slice46/1 -> reinterpret46/1
  reinterpret47/1 -> out47/1
  slice47/1 -> reinterpret47/1
  reinterpret48/1 -> out48/1
  slice48/1 -> reinterpret48/1
  reinterpret49/1 -> out49/1
  slice49/1 -> reinterpret49/1
  reinterpret50/1 -> out50/1
  slice50/1 -> reinterpret50/1
  reinterpret51/1 -> out51/1
  slice51/1 -> reinterpret51/1
  reinterpret52/1 -> out52/1
  slice52/1 -> reinterpret52/1
  reinterpret53/1 -> out53/1
  slice53/1 -> reinterpret53/1
  reinterpret54/1 -> out54/1
  slice54/1 -> reinterpret54/1
  reinterpret55/1 -> out55/1
  slice55/1 -> reinterpret55/1
  reinterpret56/1 -> out56/1
  slice56/1 -> reinterpret56/1
  reinterpret57/1 -> out57/1
  slice57/1 -> reinterpret57/1
  reinterpret58/1 -> out58/1
  slice58/1 -> reinterpret58/1
  reinterpret59/1 -> out59/1
  slice59/1 -> reinterpret59/1
  reinterpret60/1 -> out60/1
  slice60/1 -> reinterpret60/1
  reinterpret61/1 -> out61/1
  slice61/1 -> reinterpret61/1
  reinterpret62/1 -> out62/1
  slice62/1 -> reinterpret62/1
  reinterpret63/1 -> out63/1
  slice63/1 -> reinterpret63/1
  reinterpret64/1 -> out64/1
  slice64/1 -> reinterpret64/1
  reinterpret65/1 -> out65/1
  slice65/1 -> reinterpret65/1
  reinterpret66/1 -> out66/1
  slice66/1 -> reinterpret66/1
  reinterpret67/1 -> out67/1
  slice67/1 -> reinterpret67/1
  reinterpret68/1 -> out68/1
  slice68/1 -> reinterpret68/1
  reinterpret69/1 -> out69/1
  slice69/1 -> reinterpret69/1
  reinterpret70/1 -> out70/1
  slice70/1 -> reinterpret70/1
  reinterpret71/1 -> out71/1
  slice71/1 -> reinterpret71/1
  reinterpret72/1 -> out72/1
  slice72/1 -> reinterpret72/1
  reinterpret73/1 -> out73/1
  slice73/1 -> reinterpret73/1
  reinterpret74/1 -> out74/1
  slice74/1 -> reinterpret74/1
  reinterpret75/1 -> out75/1
  slice75/1 -> reinterpret75/1
  reinterpret76/1 -> out76/1
  slice76/1 -> reinterpret76/1
  reinterpret77/1 -> out77/1
  slice77/1 -> reinterpret77/1
  reinterpret78/1 -> out78/1
  slice78/1 -> reinterpret78/1
  reinterpret79/1 -> out79/1
  slice79/1 -> reinterpret79/1
  reinterpret80/1 -> out80/1
  slice80/1 -> reinterpret80/1
  reinterpret81/1 -> msb_out81/1
  slice81/1 -> reinterpret81/1
  bus_in/1 -> slice1/1, slice2/1, slice3/1, slice4/1, slice5/1, slice6/1, slice7/1, slice8/1, slice9/1, slice10/1, slice11/1, slice12/1, slice13/1, slice14/1, slice15/1, slice16/1, slice17/1, slice18/1, slice19/1, slice20/1, slice21/1, slice22/1, slice23/1, slice24/1, slice25/1, slice26/1, slice27/1, slice28/1, slice29/1, slice30/1, slice31/1, slice32/1, slice33/1, slice34/1, slice35/1, slice36/1, slice37/1, slice38/1, slice39/1, slice40/1, slice41/1, slice42/1, slice43/1, slice44/1, slice45/1, slice46/1, slice47/1, slice48/1, slice49/1, slice50/1, slice51/1, slice52/1, slice53/1, slice54/1, slice55/1, slice56/1, slice57/1, slice58/1, slice59/1, slice60/1, slice61/1, slice62/1, slice63/1, slice64/1, slice65/1, slice66/1, slice67/1, slice68/1, slice69/1, slice70/1, slice71/1, slice72/1, slice73/1, slice74/1, slice75/1, slice76/1, slice77/1, slice78/1, slice79/1, slice80/1, slice81/1
